simulink model "Robotic Vacuum Project"  (R2026a)
settings: Solver=VariableStepAuto  StopTime=100  MaxStep=0.1
InitFcn:
  | setupVacuumSimTrace;
StartFcn:
  | learning.simulink.modelCallbacks.startFunction(gcs);
StopFcn:
  | learning.simulink.modelCallbacks.stopFunction(gcs);
model workspace (MAT data in the model file):
  courseObject.course = 'stateflow'
  courseObject.chapter = 11
  courseObject.lesson = 1
  courseObject.section = 3
  courseObject.task = 1
undefined symbols (not defined in the file): axleLength, DiscIntNeverNeededParam, dockX, dockY, initialPos, robotDiam, roomHeight, roomWidth, wheelRadius
libraries: simulink x1, signalChecks x1
CloseFcn:
  | learning.simulink.cleanupOnlineTraining;learning.simulink.Application.getInstance().dduxLogMatlabEvent("ModelClosed");
  | if exist('fh','var') && fh.isvalid;close(fh);end;
  | clear('fh','ah','dockHandle','orientationHandle','traceHandle','robotHandle','closefn','existingFigures','figureName','figureTag','lineLength')
Description:
  | TrainingCourseModel
settings Model: Creator=PC  LastModifiedBy=PC

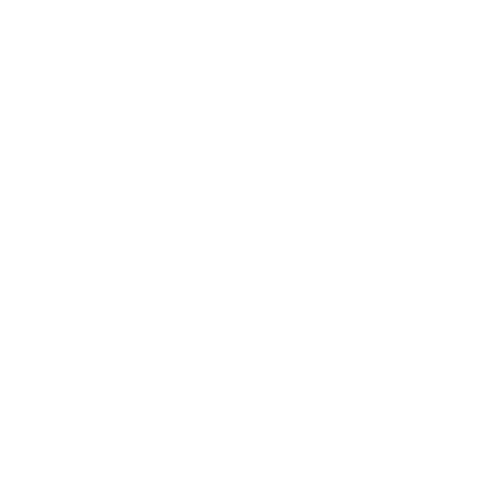
[thumbnail: Simulink's stored preview of the top-level diagram]
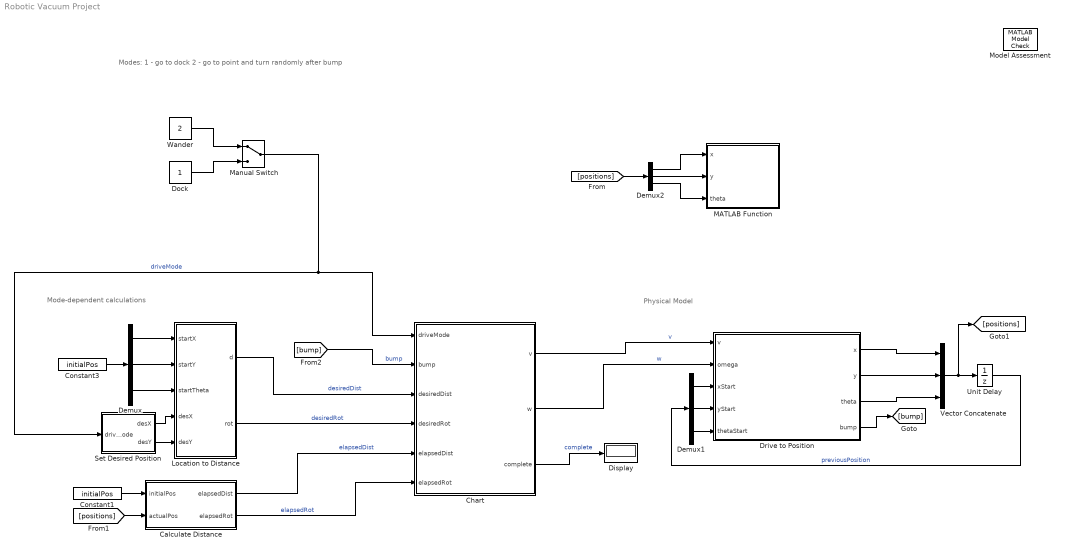
== system Robotic Vacuum Project ==
  note: Modes:
      | 1 - go to dock
      | 2 - go to point and turn randomly after bump
  note: Mode-dependent calculations
  note: Physical Model
  Calculate Distance : Subsystem
  Chart : Stateflow chart  TreatAsAtomicUnit=on
  Constant1 : Constant  Value=initialPos
  Constant3 : Constant  Value=initialPos
  Demux : Demux  Outputs=3
  Demux1 : Demux  Outputs=3
  Demux2 : Demux  Outputs=3
  Display : Display
  Dock : Constant
  Drive to Position : Subsystem
  Location to Distance : Subsystem
  MATLAB Function : MATLAB Function  TreatAsAtomicUnit=on
  Manual Switch : ManualSwitch
      settings: AttributesFormatString=(Double-click to switch modes)
  Model Assessment : signalChecks/MATLAB Model Check  mlfunc='grader_interaction2_task8'  lesson=0  task=8  pass=-1
      settings: AttributesFormatString=|
      | No input required
      | for this task
  Set Desired Position : Subsystem
  Unit Delay : UnitDelay  InitialCondition=initialPos  SampleTime=-1
  Vector Concatenate : Concatenate  NumInputs=3
  Wander : Constant  Value=2
  wires:
  Chart/2(w) -> Drive to Position/2(omega)  "w"
  Calculate Distance/1(elapsedDist) -> Chart/5(elapsedDist)  "elapsedDist"
  Location to Distance/2(rot) -> Chart/4(desiredRot)  "desiredRot"
  Chart/1(v) -> Drive to Position/1(v)  "v"
  Chart/3(complete) -> Display/1  "complete"
  Location to Distance/1(d) -> Chart/3(desiredDist)  "desiredDist"
  Constant3/1 -> Demux/1
  Set Desired Position/2(desY) -> Location to Distance/5(desY)
  [bump] -> Chart/2(bump)  "bump"
  Vector Concatenate/1 -> Unit Delay/1, [positions]
  Drive to Position/4(bump) -> [bump]
  Constant1/1 -> Calculate Distance/1(initialPos)
  Drive to Position/1(x) -> Vector Concatenate/1
  Demux1/1 -> Drive to Position/3(xStart)
  Demux1/2 -> Drive to Position/4(yStart)
  Dock/1 -> Manual Switch/2
  Wander/1 -> Manual Switch/1
  Demux/3 -> Location to Distance/3(startTheta)
  Calculate Distance/2(elapsedRot) -> Chart/6(elapsedRot)  "elapsedRot"
  Manual Switch/1 -> Chart/1(driveMode), Set Desired Position/1(driveMode)  "driveMode"
  Unit Delay/1 -> Demux1/1  "previousPosition"
  Demux1/3 -> Drive to Position/5(thetaStart)
  Set Desired Position/1(desX) -> Location to Distance/4(desX)
  Demux/1 -> Location to Distance/1(startX)
  Demux/2 -> Location to Distance/2(startY)
  Drive to Position/2(y) -> Vector Concatenate/2
  [positions] -> Demux2/1
  Drive to Position/3(theta) -> Vector Concatenate/3
  Demux2/2 -> MATLAB Function/2(y)
  Demux2/1 -> MATLAB Function/1(x)
  Demux2/3 -> MATLAB Function/3(theta)
  [positions] -> Calculate Distance/2(actualPos)

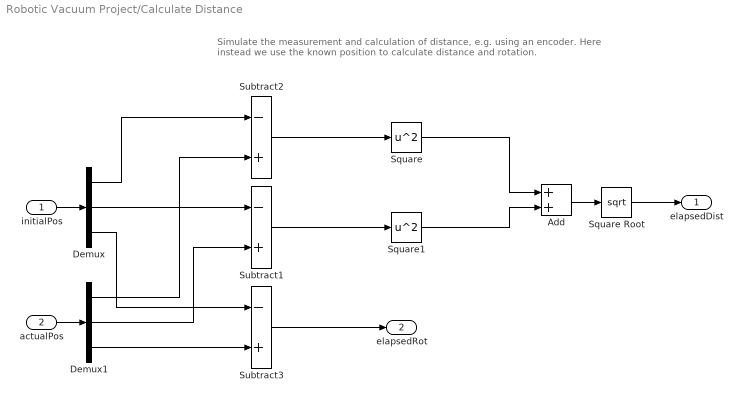
== system Robotic Vacuum Project/Calculate Distance ==
  note: Simulate the measurement and calculation of distance, e.g. using an encoder.
      | Here instead we use the known position to calculate distance and rotation.
  initialPos : Inport
  actualPos : Inport  Port=2
  Add : Sum
  Demux : Demux  Outputs=3
  Demux1 : Demux  Outputs=3
  Square : Math  Operator=square  SignedPower=on
  Square Root : Sqrt
  Square1 : Math  Operator=square  SignedPower=on
  Subtract1 : Sum  Inputs=-+
  Subtract2 : Sum  Inputs=-+
  Subtract3 : Sum  Inputs=-+
  elapsedDist : Outport  VectorParamsAs1DForOutWhenUnconnected=off
  elapsedRot : Outport  Port=2  VectorParamsAs1DForOutWhenUnconnected=off
  wires:
  actualPos/1 -> Demux1/1
  Subtract3/1 -> elapsedRot/1
  initialPos/1 -> Demux/1
  Demux/3 -> Subtract3/1
  Demux1/3 -> Subtract3/2
  Square Root/1 -> elapsedDist/1
  Add/1 -> Square Root/1
  Square1/1 -> Add/2
  Square/1 -> Add/1
  Subtract1/1 -> Square1/1
  Subtract2/1 -> Square/1
  Demux1/2 -> Subtract1/2
  Demux/2 -> Subtract1/1
  Demux1/1 -> Subtract2/2
  Demux/1 -> Subtract2/1

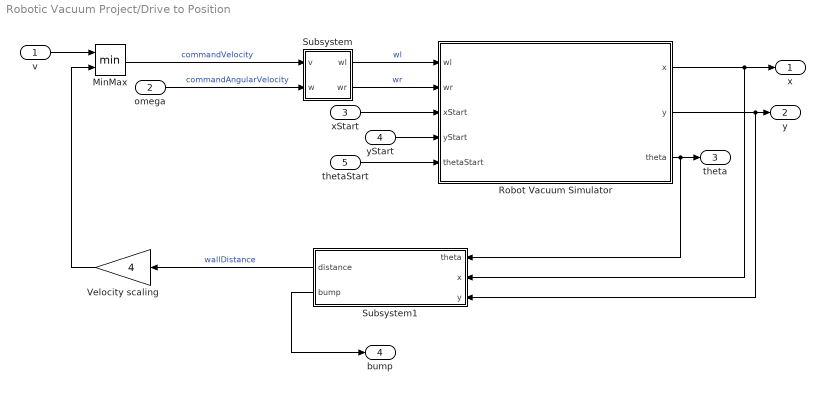
== system Robotic Vacuum Project/Drive to Position ==
  v : Inport
  omega : Inport  Port=2
  xStart : Inport  Port=3
  yStart : Inport  Port=4
  thetaStart : Inport  Port=5
  MinMax : MinMax  Inputs=2
  Robot Vacuum Simulator : Subsystem  mask(Robot Vacuum Simulator){roomW=roomWidth, roomH=roomHeight, dockX=dockX, dockY=dockY, axleLength=axleLength, wheelR=wheelRadius}
      mask prompts: roomW "Room Width (m)"; roomH "Room Height (m)"; dockX "Dock X (m)"; dockY "Dock Y (m)"; axleLength "Axle Length (m)"; wheelR "Wheel Radius (m)"
      mask help: Model a robot vacuum as a differential drive robot. Simulate its trajectory given prescribed left and right wheel rotation rates (wl, wr) and starting configuration (xStart, yStart, thetaStart).
      mask DialogControl roomProps Prompt: Room Properties
      mask DialogControl robotProps Prompt: Robot Properties
      mask Display: disp('Robot Vacuum Simulator')
  Subsystem : Subsystem  mask(Velocities to wheel angular velocities){axleLength=axleLength, wheelR=wheelRadius}
      mask prompts: axleLength "Axle Length"; wheelR "Wheel Radius"
      mask help: Converts robot linear (v) and angular (w) velocities into left (wl) and right (wr) wheel angular velocities using robot parameters.
  Subsystem1 : Subsystem  mask(Sensor Data Simulator){maxDist=2, minDist=.005}
      mask prompts: maxDist "Maximum sensing distance (m)"; minDist "Minimum sensing distance (m)"
      mask help: Simulate the sensor data from two sensors: an ultrasonic distance sensor measuring distance in meters, and a bump sensor that outputs one when the robot bumps into a wall.
      mask DialogControl Container3 Prompt: Ultrasonic Sensor Properties
      mask Display: disp('Sensor Data Simulator');
  Velocity scaling : Gain  Gain=4
  x : Outport
  y : Outport  Port=2
  theta : Outport  Port=3
  bump : Outport  Port=4  VectorParamsAs1DForOutWhenUnconnected=off
  wires:
  Robot Vacuum Simulator/3(theta) -> theta/1, Subsystem1/1(theta)
  Robot Vacuum Simulator/2(y) -> y/1, Subsystem1/3(y)
  Robot Vacuum Simulator/1(x) -> x/1, Subsystem1/2(x)
  Subsystem1/2(bump) -> bump/1
  v/1 -> MinMax/1
  MinMax/1 -> Subsystem/1(v)  "commandVelocity"
  thetaStart/1 -> Robot Vacuum Simulator/5(thetaStart)
  yStart/1 -> Robot Vacuum Simulator/4(yStart)
  xStart/1 -> Robot Vacuum Simulator/3(xStart)
  Subsystem/2(wr) -> Robot Vacuum Simulator/2(wr)  "wr"
  Subsystem/1(wl) -> Robot Vacuum Simulator/1(wl)  "wl"
  Subsystem1/1(distance) -> Velocity scaling/1  "wallDistance"
  omega/1 -> Subsystem/2(w)  "commandAngularVelocity"
  Velocity scaling/1 -> MinMax/2

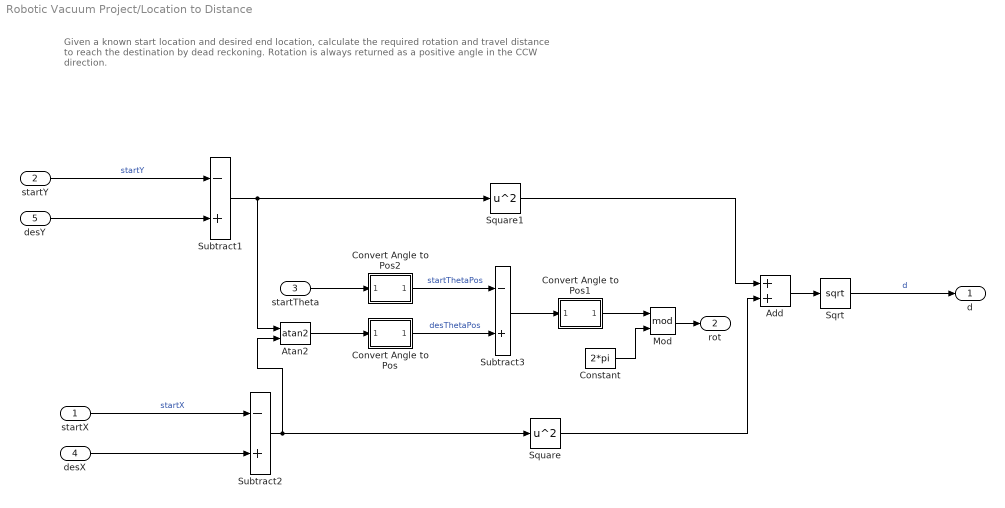
== system Robotic Vacuum Project/Location to Distance ==
  note: Given a known start location and desired end location, calculate the required rotation and travel distance to reach the destination by dead reckoning.
      | Rotation is always returned as a positive angle in the CCW direction.
  startX : Inport
  startY : Inport  Port=2
  startTheta : Inport  Port=3
  desX : Inport  Port=4
  desY : Inport  Port=5
  Add : Sum
  Atan2 : Trigonometry  Operator=atan2
  Constant : Constant  Value=2*pi
  Convert Angle to Pos : Subsystem
  Convert Angle to Pos1 : Subsystem
  Convert Angle to Pos2 : Subsystem
  Mod : Math  Operator=mod
  Sqrt : Sqrt
  Square : Math  Operator=square  SignedPower=on
  Square1 : Math  Operator=square  SignedPower=on
  Subtract1 : Sum  Inputs=-+
  Subtract2 : Sum  Inputs=-+
  Subtract3 : Sum  Inputs=-+
  d : Outport  VectorParamsAs1DForOutWhenUnconnected=off
  rot : Outport  Port=2  VectorParamsAs1DForOutWhenUnconnected=off
  wires:
  Constant/1 -> Mod/2
  Mod/1 -> rot/1
  Convert Angle to Pos2/1(Out1) -> Subtract3/1  "startThetaPos"
  Convert Angle to Pos/1(Out1) -> Subtract3/2  "desThetaPos"
  Atan2/1 -> Convert Angle to Pos/1(In1)
  Subtract3/1 -> Convert Angle to Pos1/1(In1)
  Convert Angle to Pos1/1(Out1) -> Mod/1
  startTheta/1 -> Convert Angle to Pos2/1(In1)
  Sqrt/1 -> d/1  "d"
  Add/1 -> Sqrt/1
  Square1/1 -> Add/1
  Square/1 -> Add/2
  Subtract1/1 -> Square1/1, Atan2/1
  Subtract2/1 -> Square/1, Atan2/2
  desY/1 -> Subtract1/2
  startY/1 -> Subtract1/1  "startY"
  desX/1 -> Subtract2/2
  startX/1 -> Subtract2/1  "startX"

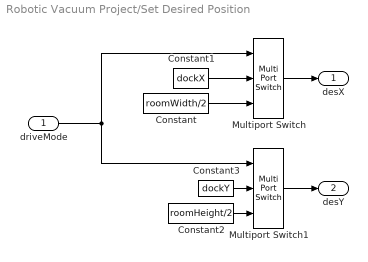
== system Robotic Vacuum Project/Set Desired Position ==
  driveMode : Inport
  Constant : Constant  Value=roomWidth/2
  Constant1 : Constant  Value=dockX
  Constant2 : Constant  Value=roomHeight/2
  Constant3 : Constant  Value=dockY
  Multiport Switch : MultiPortSwitch  Inputs=2  SaturateOnIntegerOverflow=off  InputSameDT=off
  Multiport Switch1 : MultiPortSwitch  Inputs=2  SaturateOnIntegerOverflow=off  InputSameDT=off
  desX : Outport  VectorParamsAs1DForOutWhenUnconnected=off
  desY : Outport  Port=2  VectorParamsAs1DForOutWhenUnconnected=off
  wires:
  Multiport Switch1/1 -> desY/1
  Constant3/1 -> Multiport Switch1/2
  Constant2/1 -> Multiport Switch1/3
  Constant/1 -> Multiport Switch/3
  Constant1/1 -> Multiport Switch/2
  driveMode/1 -> Multiport Switch1/1, Multiport Switch/1
  Multiport Switch/1 -> desX/1

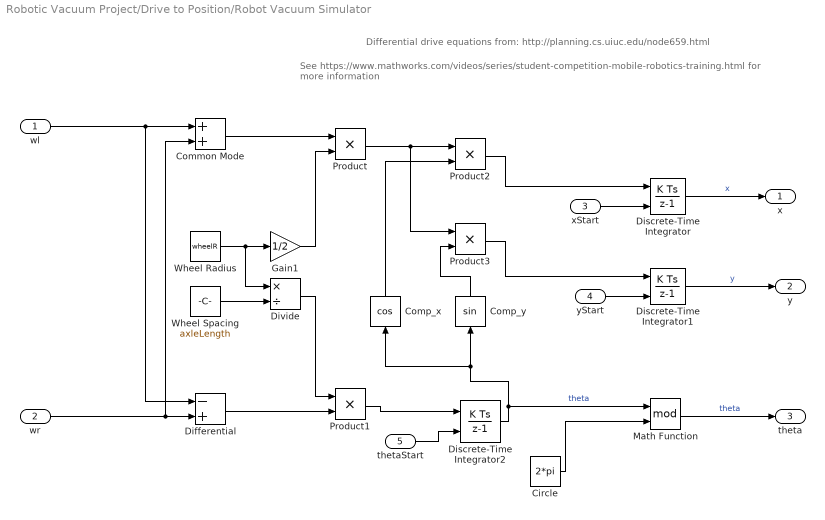
== system Robotic Vacuum Project/Drive to Position/Robot Vacuum Simulator ==
  note: See https://www.mathworks.com/videos/series/student-competition-mobile-robotics-training.html for more information
  note: Differential drive equations from: http://planning.cs.uiuc.edu/node659.html
  wl : Inport
  wr : Inport  Port=2
  xStart : Inport  Port=3
  yStart : Inport  Port=4
  thetaStart : Inport  Port=5
  Circle : Constant  Value=2*pi
  Common Mode : Sum
  Comp_x : Trigonometry  Operator=cos
  Comp_y : Trigonometry
  Differential : Sum  Inputs=-+
  Discrete-Time Integrator : DiscreteIntegrator  InitialConditionSource=external  SampleTime=-1  ICPrevOutput=DiscIntNeverNeededParam  ICPrevScaledInput=DiscIntNeverNeededParam
  Discrete-Time Integrator1 : DiscreteIntegrator  InitialConditionSource=external  SampleTime=-1  ICPrevOutput=DiscIntNeverNeededParam  ICPrevScaledInput=DiscIntNeverNeededParam
  Discrete-Time Integrator2 : DiscreteIntegrator  InitialConditionSource=external  SampleTime=-1  ICPrevOutput=DiscIntNeverNeededParam  ICPrevScaledInput=DiscIntNeverNeededParam
  Divide : Product  Inputs=*/
  Gain1 : Gain  Gain=1/2
  Math Function : Math  Operator=mod  SignedPower=on
  Product{,1..3} (4 alike) : Product  RndMeth=Zero
  Wheel Radius : Constant  Value=wheelR
  Wheel Spacing : Constant  Value=axleLength
  x : Outport
  y : Outport  Port=2
  theta : Outport  Port=3
  wires:
  yStart/1 -> Discrete-Time Integrator1/2
  xStart/1 -> Discrete-Time Integrator/2
  thetaStart/1 -> Discrete-Time Integrator2/2
  Common Mode/1 -> Product/1
  Circle/1 -> Math Function/2
  Differential/1 -> Product1/2
  Math Function/1 -> theta/1  "theta"
  Wheel Radius/1 -> Gain1/1, Divide/1
  wr/1 -> Differential/2, Common Mode/2
  Comp_y/1 -> Product3/2
  Product2/1 -> Discrete-Time Integrator/1
  Product/1 -> Product2/1, Product3/1
  Gain1/1 -> Product/2
  Product1/1 -> Discrete-Time Integrator2/1
  Wheel Spacing/1 -> Divide/2
  Discrete-Time Integrator1/1 -> y/1  "y"
  Discrete-Time Integrator/1 -> x/1  "x"
  Comp_x/1 -> Product2/2
  Product3/1 -> Discrete-Time Integrator1/1
  wl/1 -> Differential/1, Common Mode/1
  Discrete-Time Integrator2/1 -> Comp_y/1, Comp_x/1, Math Function/1  "theta"
  Divide/1 -> Product1/1

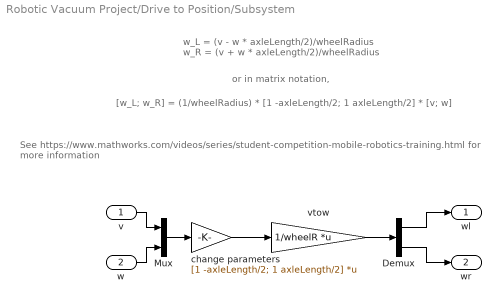
== system Robotic Vacuum Project/Drive to Position/Subsystem ==
  note: or in matrix notation,
  note: w_L  = (v - w * axleLength/2)/wheelRadius
      | w_R = (v + w * axleLength/2)/wheelRadius
  note: [w_L; w_R] = (1/wheelRadius) * [1 -axleLength/2; 1 axleLength/2] * [v; w]
  note: See https://www.mathworks.com/videos/series/student-competition-mobile-robotics-training.html for more information
  v : Inport
  w : Inport  Port=2
  Demux : Demux  Outputs=2
  Mux : Mux  Inputs=2
  change parameters : Gain  Gain=[1 -axleLength/2; 1 axleLength/2]  Multiplication=Matrix(K*u)
  vtow : Gain  Gain=1/wheelR  Multiplication=Matrix(K*u)
  wl : Outport  VectorParamsAs1DForOutWhenUnconnected=off
  wr : Outport  Port=2  VectorParamsAs1DForOutWhenUnconnected=off
  wires:
  Mux/1 -> change parameters/1
  Demux/2 -> wr/1
  Demux/1 -> wl/1
  v/1 -> Mux/1
  vtow/1 -> Demux/1
  w/1 -> Mux/2
  change parameters/1 -> vtow/1

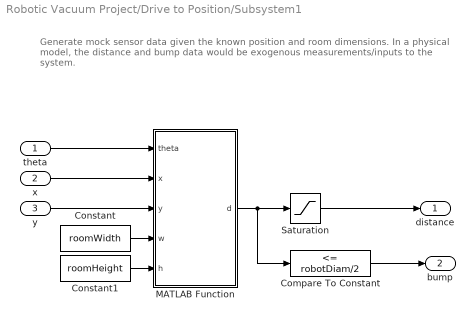
== system Robotic Vacuum Project/Drive to Position/Subsystem1 ==
  note: Generate mock sensor data given the known position and room dimensions.
      | In a physical model, the distance and bump data would be exogenous
      | measurements/inputs to the system.
  theta : Inport
  x : Inport  Port=2
  y : Inport  Port=3
  Compare To Constant : simulink/Logic and Bit Operations/Compare To Constant  relop=<=  const=robotDiam/2  OutDataTypeStr=boolean
  Constant : Constant  Value=roomWidth
  Constant1 : Constant  Value=roomHeight
  MATLAB Function : MATLAB Function  TreatAsAtomicUnit=on
  Saturation : Saturate  UpperLimit=maxDist  LowerLimit=minDist
  distance : Outport  VectorParamsAs1DForOutWhenUnconnected=off
  bump : Outport  Port=2  VectorParamsAs1DForOutWhenUnconnected=off
  wires:
  Compare To Constant/1 -> bump/1
  MATLAB Function/1(d) -> Saturation/1, Compare To Constant/1
  Saturation/1 -> distance/1
  y/1 -> MATLAB Function/3(y)
  x/1 -> MATLAB Function/2(x)
  theta/1 -> MATLAB Function/1(theta)
  Constant/1 -> MATLAB Function/4(w)
  Constant1/1 -> MATLAB Function/5(h)

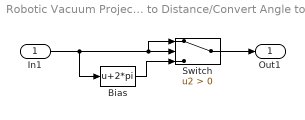
== system Robotic Vacuum Project/Location to Distance/Convert Angle to Pos ==
  In1 : Inport
  Bias : Bias  Bias=2*pi  SaturateOnIntegerOverflow=off
  Switch : Switch  Criteria=u2 > Threshold  SaturateOnIntegerOverflow=off  InputSameDT=off
  Out1 : Outport  VectorParamsAs1DForOutWhenUnconnected=off
  wires:
  Bias/1 -> Switch/3
  Switch/1 -> Out1/1
  In1/1 -> Switch/1, Switch/2, Bias/1

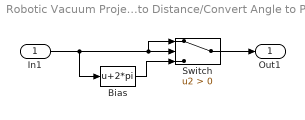
== system Robotic Vacuum Project/Location to Distance/Convert Angle to Pos1 ==
  In1 : Inport
  Bias : Bias  Bias=2*pi  SaturateOnIntegerOverflow=off
  Switch : Switch  Criteria=u2 > Threshold  SaturateOnIntegerOverflow=off  InputSameDT=off
  Out1 : Outport  VectorParamsAs1DForOutWhenUnconnected=off
  wires:
  Bias/1 -> Switch/3
  Switch/1 -> Out1/1
  In1/1 -> Switch/1, Switch/2, Bias/1

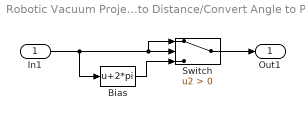
== system Robotic Vacuum Project/Location to Distance/Convert Angle to Pos2 ==
  In1 : Inport
  Bias : Bias  Bias=2*pi  SaturateOnIntegerOverflow=off
  Switch : Switch  Criteria=u2 > Threshold  SaturateOnIntegerOverflow=off  InputSameDT=off
  Out1 : Outport  VectorParamsAs1DForOutWhenUnconnected=off
  wires:
  In1/1 -> Bias/1, Switch/2, Switch/1
  Switch/1 -> Out1/1
  Bias/1 -> Switch/3

== stateflow chart Robotic Vacuum Project/Chart ==
  settings: sampleTime=0.2
  state DriveToLocation
    entry:
    positionReached = 0;
    state PureRotate
      entry:
      v = 0;
      w = 1;
    state PureTranslate
      entry:
      v = 3;
      w = 0;
    state Stop
      entry:
      v = 0;
      w = 0;
      positionReached =1;
    (default) -> PureRotate
    PureRotate -> PureTranslate : [mod(elapsedDist,2*pi) >= elapsedRot]
    PureTranslate -> Stop : [desiredRot >= desiredDist]
  state TaskComplete
    entry:
    complete = 1;
  state RandomDrive
    entry:
    bumpCount = 0;
    state RotateRandom
      entry:
      v = 0;
      w = 1;
      tRotate = rand(1)*1.5+2.5;
    state FindWall
      entry:
      v = 3;
      w = 0;
    (default) -> FindWall
    FindWall -> RotateRandom : [bump == 1]{bumpCount = bumpCount + 1;}
    RotateRandom -> FindWall : after(tRotate,sec)
  (default) -> DriveToLocation
  DriveToLocation -> TaskComplete [order 1] : [driveMode == 1 && positionReached == 1]
  RandomDrive -> TaskComplete : [bumpCount > 50]
  DriveToLocation -> RandomDrive [order 2] : [driveMode == 2 && positionReached == 1]
  data: positionReached local; driveMode input; bump input; bumpCount local; v output; w output; desiredDist input; desiredRot input; elapsedDist input; elapsedRot input; tRotate local; complete output

== matlab function Robotic Vacuum Project/Drive to Position/Subsystem1/MATLAB Function ==
  data: theta input; x input; d output; y input; w input; h input
function d = distanceToWall(theta,x,y,w,h)

% Determine distance by consider direction facing and closest wall

if theta <= pi/2
    dx = w-x;
    dy = h-y;
elseif theta <= pi
    dx = x;
    dy = h-y;
elseif theta <= 3*pi/2
    dx = x;
    dy = y;
else
    dx = w-x;
    dy = y;
end

d = min([dx,dy]);

== matlab function Robotic Vacuum Project/MATLAB Function ==
  data: x input; y input; theta input
function plotRobot(x,y,theta)

coder.extrinsic('evalin','plot','isgraphics');

lineLength = .2;

oH = evalin('base','orientationHandle');
rH = evalin('base','robotHandle');
tH = evalin('base','traceHandle');

if ~isgraphics(tH) || ~isgraphics(rH) || ~isgraphics(oH)
    return
end

traceX = get(tH,'xdata');
traceY = get(tH,'ydata');

% Find length orientation line
xp = [x x+lineLength*cos(theta)];
yp = [y y+lineLength*sin(theta)];

traceX = [x traceX];
traceY = [y traceY];

% Plot robot
set(oH,'xdata',xp,'ydata',yp);
set(rH,'xdata',x,'ydata',y);
set(tH,'xdata',traceX,'ydata',traceY);
drawnow('limitrate')
